simulink model "tg9"  (R2022a)
settings: Solver=ode15s  StartTime=0.0  StopTime=10  MaxStep=0.01  RelTol=1e-3
InitFcn:
  | mecha_param2
  | control_param0
values from neighbouring files (symbols this model uses):
  b0 = 0    [sim_IMMC.m]
  b1 = 1    [sim_IMMC.m]
  back0 = 0    [sim_IMMC.m]
  back1 = 0    [sim_IMMC.m]
  boff = 0    [sim_IMMC.m]
  bon = 0    [sim_IMMC.m]
  c = 0.05    [mecha_param2.m]
  c_jointstop = 0.3 / (pi/180)    (= 17.1887338539)    [mecha_param2.m]
  calctalus = sqrt((L_foot - (DJ1x_foot))^2 + (H_foot-r_cs)^2)    [mecha_param2.m]
  calctoes = sqrt((H_foot-r_cs)^2 + (DJ1x_foot)^2)    [mecha_param2.m]
  corrD = 0.001    [control_param0.m]
  DG_HAT = 0.35    [mecha_param2.m]
  DG_thigh = 0.28    [mecha_param2.m]
  DJ1x_foot = 0.16-r_cs    (= 0.135)    [mecha_param2.m]
  eref = 0.04    [mecha_param2.m]
  FmaxBFSH = 350    [mecha_param2.m]
  FmaxGAS = 1500    [mecha_param2.m]
  FmaxGLU = 1500    [mecha_param2.m]
  FmaxHAM = 3000    [mecha_param2.m]
  FmaxHFL = 2000    [mecha_param2.m]
  FmaxRF = 1200    [mecha_param2.m]
  FmaxSOL = 4000    [mecha_param2.m]
  FmaxTA = 800    [mecha_param2.m]
  FmaxVAS = 6000    [mecha_param2.m]
  g = 9.81    [mecha_param2.m]
  g0 = 0    [sim_IMMC.m]
  g1 = 0    [sim_IMMC.m]
  H_foot = 0.08    [mecha_param2.m]
  In_HAT = 3    [mecha_param2.m]
  In_shank = 0.05    [mecha_param2.m]
  In_thigh = 0.15    [mecha_param2.m]
  K = 5    [mecha_param2.m]
  knee_thigh = [0 0 -(L_thigh/2)]    [mecha_param2.m]
  Kpress = m_HAT * g / DeltaThRef    (= 104967)    [mecha_param2.m]
  L_foot = 0.2    [mecha_param2.m]
  L_HAT = 0.8    [mecha_param2.m]
  L_shank = 0.46    [mecha_param2.m]
  L_thigh = 0.46    [mecha_param2.m]
  LoHAM = table2array(mt('LoHAM', 1))    [control_param0.m]
  LoHFL = table2array(mt('LoHFL', 1))    [control_param0.m]
  longD = longD - corrD    (= 0.019)    [control_param0.m]
  loptBFSH = 0.12    [mecha_param2.m]
  loptGAS = 0.05    [mecha_param2.m]
  loptGLU = 0.11    [mecha_param2.m]
  loptHAM = 0.10    (= 0.1)    [mecha_param2.m]
  loptHFL = 0.11    [mecha_param2.m]
  loptRF = 0.08    [mecha_param2.m]
  loptSOL = 0.04    [mecha_param2.m]
  loptTA = 0.06    [mecha_param2.m]
  loptVAS = 0.08    [mecha_param2.m]
  LoTA = table2array(mt('LoTA', 1))    [control_param0.m]
  lslackBFSH = 0.10    (= 0.1)    [mecha_param2.m]
  lslackGAS = 0.40    (= 0.4)    [mecha_param2.m]
  lslackGLU = 0.13    [mecha_param2.m]
  lslackHAM = 0.31    [mecha_param2.m]
  lslackHFL = 0.10    (= 0.1)    [mecha_param2.m]
  lslackRF = 0.35    [mecha_param2.m]
  lslackSOL = 0.26    [mecha_param2.m]
  lslackTA = 0.24    [mecha_param2.m]
  lslackVAS = 0.23    [mecha_param2.m]
  m_HAT = 53.5    [mecha_param2.m]
  m_shank = 3.5    [mecha_param2.m]
  m_thigh = 8.5    [mecha_param2.m]
  midD = midD - corrD    (= 0.009)    [control_param0.m]
  N = 1.5    [mecha_param2.m]
  nonoff = 0    [control_param0.m]
  phi_a_low = (70) * (pi / 180)    (= 1.2217304764)    [mecha_param2.m]
  phi_a_up = (130) * (pi / 180)    (= 2.26892802759)    [mecha_param2.m]
  phi_dl = 180    [mecha_param2.m]
  phi_h = 230 * (pi / 180)    (= 4.01425727959)    [mecha_param2.m]
  phi_k = 175 * (pi / 180)    (= 3.05432619099)    [mecha_param2.m]
  phictoes = asind((DJ1y_foot-r_cs)/calctoes)    [mecha_param2.m]
  phimaxGASa = 100*pi/180    (= 1.74532925199)    [mecha_param2.m]
  phimaxGASk = 140*pi/180    (= 2.44346095279)    [mecha_param2.m]
  phimaxRFk = 165*pi/180    (= 2.87979326579)    [mecha_param2.m]
  phimaxSOL = 100*pi/180    (= 1.74532925199)    [mecha_param2.m]
  phimaxTA = 80*pi/180    (= 1.3962634016)    [mecha_param2.m]
  phimaxVAS = 165*pi/180    (= 2.87979326579)    [mecha_param2.m]
  phirefBFSH = 160*pi/180    (= 2.79252680319)    [mecha_param2.m]
  phirefGASa = 80*pi/180    (= 1.3962634016)    [mecha_param2.m]
  phirefGASk = 165*pi/180    (= 2.87979326579)    [mecha_param2.m]
  phirefGLU = 120*pi/180    (= 2.09439510239)    [mecha_param2.m]
  phirefHAMh = 150*pi/180    (= 2.61799387799)    [mecha_param2.m]
  phirefHAMk = 180*pi/180    (= 3.14159265359)    [mecha_param2.m]
  phirefHFL = 160*pi/180    (= 2.79252680319)    [mecha_param2.m]
  phirefRFh = 170*pi/180    (= 2.96705972839)    [mecha_param2.m]
  phirefRFk = 125*pi/180    (= 2.18166156499)    [mecha_param2.m]
  phirefSOL = 90*pi/180    (= 1.57079632679)    [mecha_param2.m]
  phirefTA = 110*pi/180    (= 1.91986217719)    [mecha_param2.m]
  phirefVAS = 120*pi/180    (= 2.09439510239)    [mecha_param2.m]
  phiScaleGASa = acos(rGASamin/rGASamax)/(phiminGASa-phimaxGASa)    [mecha_param2.m]
  phiScaleGASk = acos(rGASkmin/rGASkmax)/(phiminGASk-phimaxGASk)    [mecha_param2.m]
  phiScaleRFk = acos(rRFkmin/rRFkmax)/(phiminRFk-phimaxRFk)    [mecha_param2.m]
  phiScaleSOL = acos(rSOLmin/rSOLmax)/(phiminSOL-phimaxSOL)    [mecha_param2.m]
  phiScaleTA = acos(rTAmin/rTAmax)/(phiminTA-phimaxTA)    [mecha_param2.m]
  phiScaleVAS = acos(rVASmin/rVASmax)/(phiminVAS-phimaxVAS)    [mecha_param2.m]
  r1 = 0    [sim_IMMC.m]
  r_cs = 0.025    [mecha_param2.m]
  rBFSH = 0.04    [mecha_param2.m]
  rGASamax = 0.06    [mecha_param2.m]
  rGASkmax = 0.05    [mecha_param2.m]
  rGLU = 0.08    [mecha_param2.m]
  rHAMh = 0.08    [mecha_param2.m]
  rHAMk = 0.05    [mecha_param2.m]
  rHFL = 0.08    [mecha_param2.m]
  rhoBFSH = 0.7    [mecha_param2.m]
  rhoGASa = 0.7    [mecha_param2.m]
  rhoGASk = 0.7    [mecha_param2.m]
  rhoGLU = 0.5    [mecha_param2.m]
  rhoHAMh = 0.5    [mecha_param2.m]
  rhoHAMk = 0.5    [mecha_param2.m]
  rhoHFL = 0.5    [mecha_param2.m]
  rhoRFh = 0.3    [mecha_param2.m]
  rhoRFk = 0.5    [mecha_param2.m]
  rhoSOL = 0.5    [mecha_param2.m]
  rhoTA = 0.7    [mecha_param2.m]
  rhoVAS = 0.6    [mecha_param2.m]
  rRFh = 0.08    [mecha_param2.m]
  rRFkmax = 0.06    [mecha_param2.m]
  rSOLmax = 0.06    [mecha_param2.m]
  ... (+25 more)
undefined symbols (not defined in the file or in its folder): beta11, beta12, beta13, beta14, beta15, beta16, beta21, beta22, beta23, beta24, beta25, beta26, beta31, beta32, beta33, beta34, beta35, beta36, beta41, beta42, beta43, beta44, beta45, beta46, beta51, beta52, beta53, beta54, beta55, beta56, betab1, betab2, betab3, betab4, betab5, betab6, betap11, betap12, betap13, betap14, betap15, betap16, betap21, betap22, betap23, betap24, betap25, betap26, betap31, betap32, betap33, betap34, betap35, betap36, betap41, betap42, betap43, betap44, betap45, betap46 ... (+102)
libraries: sm_lib x89, simulink x72, nesl_utility x58, simulink_extras x18
(part 9 of 12)

== system tg9/Muscle Actuation Layer/L GLU/CE inverse force-velocity relation ==
  note: u(1) * (u(2)<=1)
  note: CE, inverse force-velocity relationship
  note: K*fv
  note: 1+K*fv
  note: fv-1
  Fv[Fmax] : Inport
  Constant{,1,3..4} (4 alike) : Constant
  Constant2 : Constant  Value=N
  Constant5 : Constant  Value=N
  Divide2 : Product  Inputs=/*
  Divide3 : Product  Inputs=*/
  Gain : Gain  Gain=K
  Gain2 : Gain  Gain=7.56*K
  Gain3 : Gain  Gain=1e-2
  Mux : Mux  Inputs=3
  Mux1 : Mux  Inputs=2
  Mux2 : Mux  Inputs=3
  Product : Product  Inputs=*/
  Sum : Sum  Inputs=|+-
  Sum1 : Sum  Inputs=++|
  Sum2 : Sum  Inputs=+|+
  Sum3 : Sum  Inputs=+|+
  Sum4 : Sum  Inputs=-+|
  Sum5 : Sum  Inputs=|-+
  Sum6 : Sum  Inputs=|++
  Sum7 : Sum  Inputs=+-|
  Sum8 : Sum  Inputs=|++
  excentric branch1 : Fcn  Expr=u(2) * (u(1)>1)*(u(1)<=u(3))
  excentric branch2 : Fcn  Expr=u(1) * (u(2)<=1)
  excentric branch3 : Fcn  Expr=u(3) * (u(2)>u(1))
  v[vmax] : Outport
  wires:
  Sum/1 -> Product/1
  Constant1/1 -> Sum/2, Sum1/1
  Gain/1 -> Sum1/2
  Sum1/1 -> Product/2
  Product/1 -> Mux1/1
  Mux1/1 -> excentric branch2/1
  excentric branch2/1 -> Sum3/1
  Sum3/1 -> v[vmax]/1
  Constant2/1 -> Sum5/2, Sum4/1
  Constant3/1 -> Sum5/1
  Sum5/1 -> Divide2/1
  Sum4/1 -> Gain3/1, Divide2/2
  Sum6/1 -> Divide3/1
  Constant/1 -> Sum7/1, Sum6/2
  Divide2/1 -> Gain2/1, Sum6/1
  Sum7/1 -> Divide3/2
  Gain2/1 -> Sum7/2
  Gain3/1 -> Sum8/1
  Constant4/1 -> Sum8/2
  Sum8/1 -> Mux/3
  Divide3/1 -> Mux2/2
  Constant5/1 -> Mux/1, Mux2/3
  Mux2/1 -> excentric branch1/1
  Mux/1 -> excentric branch3/1
  excentric branch1/1 -> Sum2/1
  excentric branch3/1 -> Sum2/2
  Sum2/1 -> Sum3/2
  Fv[Fmax]/1 -> Mux/2, Mux2/1, Mux1/2, Gain/1, Sum/1, Sum4/2

== system tg9/Muscle Actuation Layer/L GLU/PE force-length relation ==
  note: tendon reference strain, relative to lslack
  note: if lse > 1
  note: lce-1
  note: ((lce-1)/w)^2
  note: fpe, force-length relationship
  lce [lopt] : Inport
  Constant : Constant  Value=w
  Constant1 : Constant
  Math Function : Math  Operator=square
  Mux : Mux  Inputs=2
  Sum : Sum  Inputs=|+-
  excentric branch1 : Fcn  Expr=u(2) * (u(1)>1)
  relative strain : Product  Inputs=*/
  fpe [Fmax] : Outport
  wires:
  excentric branch1/1 -> fpe [Fmax]/1
  Mux/1 -> excentric branch1/1
  relative strain/1 -> Math Function/1
  Constant1/1 -> Sum/2
  Sum/1 -> relative strain/1
  lce [lopt]/1 -> Mux/1, Sum/1
  Constant/1 -> relative strain/2
  Math Function/1 -> Mux/2

== system tg9/Muscle Actuation Layer/L GLU/SE force-length relation ==
  note: fse, elastic force-length relationship
  note: tendon reference strain, relative to lslack
  note: e = (lse-lslack)/lslack;
      | e = lse[lslack]-1
  note: (e/eref)^2
  note: e>0 or lse>1
  lse [lslack] : Inport
  Constant : Constant  Value=eref
  Constant1 : Constant
  Math Function : Math  Operator=square
  Mux : Mux  Inputs=2
  Sum : Sum  Inputs=|+-
  excentric branch1 : Fcn  Expr=u(2)*(u(1)>1)
  relative strain : Product  Inputs=*/
  fse [Fmax] : Outport
  wires:
  lse [lslack]/1 -> Mux/1, Sum/1
  Sum/1 -> relative strain/1
  Constant1/1 -> Sum/2
  Constant/1 -> relative strain/2
  relative strain/1 -> Math Function/1
  Math Function/1 -> Mux/2
  Mux/1 -> excentric branch1/1
  excentric branch1/1 -> fse [Fmax]/1

== system tg9/Muscle Actuation Layer/L HAM/BE force-length relation ==
  note: reference compression
  note: if lce<1-w
  note: lce[lopt]-(1-w)
  note: ((lce+w-1)/(w/2))^2
  note: fbe, compression force-length relationship
  lce [lopt] : Inport
  Constant : Constant  Value=w/2
  Constant1 : Constant  Value=1-w
  Math Function : Math  Operator=square
  Mux : Mux  Inputs=2
  Sum : Sum  Inputs=|+-
  excentric branch1 : Fcn  Expr=u(2)*(u(1)<0)
  relative strain : Product  Inputs=*/
  fbe [Fmax] : Outport
  wires:
  excentric branch1/1 -> fbe [Fmax]/1
  Mux/1 -> excentric branch1/1
  relative strain/1 -> Math Function/1
  Constant1/1 -> Sum/2
  Sum/1 -> Mux/1, relative strain/1
  lce [lopt]/1 -> Sum/1
  Constant/1 -> relative strain/2
  Math Function/1 -> Mux/2

== system tg9/Muscle Actuation Layer/L HAM/CE force-length relation ==
  note: fce, force-length relationship
  note: lce-1
  note: |lce-1|
  note: |lce-1|/w
  note: (|lce-1|/w)^3
  lce [lopt] : Inport
  Abs : Abs  SaturateOnIntegerOverflow=off
  Constant : Constant
  Constant1 : Constant  Value=w
  Constant2 : Constant  Value=3
  Exp : Math
  Exp1 : Math  Operator=pow  SignedPower=on
  Gain : Gain  Gain=log(c)
  Sum : Sum  Inputs=|+-
  normalized position : Product  Inputs=*/
  fce [Fmax] : Outport
  wires:
  lce [lopt]/1 -> Sum/1
  Constant/1 -> Sum/2
  Constant1/1 -> normalized position/2
  Sum/1 -> Abs/1
  Abs/1 -> normalized position/1
  normalized position/1 -> Exp1/1
  Constant2/1 -> Exp1/2
  Exp1/1 -> Gain/1
  Gain/1 -> Exp/1
  Exp/1 -> fce [Fmax]/1

== system tg9/Muscle Actuation Layer/L HAM/CE inverse force-velocity relation ==
  note: u(1) * (u(2)<=1)
  note: CE, inverse force-velocity relationship
  note: K*fv
  note: 1+K*fv
  note: fv-1
  Fv[Fmax] : Inport
  Constant{,1,3..4} (4 alike) : Constant
  Constant2 : Constant  Value=N
  Constant5 : Constant  Value=N
  Divide2 : Product  Inputs=/*
  Divide3 : Product  Inputs=*/
  Gain : Gain  Gain=K
  Gain2 : Gain  Gain=7.56*K
  Gain3 : Gain  Gain=1e-2
  Mux : Mux  Inputs=3
  Mux1 : Mux  Inputs=2
  Mux2 : Mux  Inputs=3
  Product : Product  Inputs=*/
  Sum : Sum  Inputs=|+-
  Sum1 : Sum  Inputs=++|
  Sum2 : Sum  Inputs=+|+
  Sum3 : Sum  Inputs=+|+
  Sum4 : Sum  Inputs=-+|
  Sum5 : Sum  Inputs=|-+
  Sum6 : Sum  Inputs=|++
  Sum7 : Sum  Inputs=+-|
  Sum8 : Sum  Inputs=|++
  excentric branch1 : Fcn  Expr=u(2) * (u(1)>1)*(u(1)<=u(3))
  excentric branch2 : Fcn  Expr=u(1) * (u(2)<=1)
  excentric branch3 : Fcn  Expr=u(3) * (u(2)>u(1))
  v[vmax] : Outport
  wires:
  Sum/1 -> Product/1
  Constant1/1 -> Sum/2, Sum1/1
  Gain/1 -> Sum1/2
  Sum1/1 -> Product/2
  Product/1 -> Mux1/1
  Mux1/1 -> excentric branch2/1
  excentric branch2/1 -> Sum3/1
  Sum3/1 -> v[vmax]/1
  Constant2/1 -> Sum5/2, Sum4/1
  Constant3/1 -> Sum5/1
  Sum5/1 -> Divide2/1
  Sum4/1 -> Gain3/1, Divide2/2
  Sum6/1 -> Divide3/1
  Constant/1 -> Sum7/1, Sum6/2
  Divide2/1 -> Gain2/1, Sum6/1
  Sum7/1 -> Divide3/2
  Gain2/1 -> Sum7/2
  Gain3/1 -> Sum8/1
  Constant4/1 -> Sum8/2
  Sum8/1 -> Mux/3
  Divide3/1 -> Mux2/2
  Constant5/1 -> Mux/1, Mux2/3
  Mux2/1 -> excentric branch1/1
  Mux/1 -> excentric branch3/1
  excentric branch1/1 -> Sum2/1
  excentric branch3/1 -> Sum2/2
  Sum2/1 -> Sum3/2
  Fv[Fmax]/1 -> Mux/2, Mux2/1, Mux1/2, Gain/1, Sum/1, Sum4/2

== system tg9/Muscle Actuation Layer/L HAM/PE force-length relation ==
  note: tendon reference strain, relative to lslack
  note: if lse > 1
  note: lce-1
  note: ((lce-1)/w)^2
  note: fpe, force-length relationship
  lce [lopt] : Inport
  Constant : Constant  Value=w
  Constant1 : Constant
  Math Function : Math  Operator=square
  Mux : Mux  Inputs=2
  Sum : Sum  Inputs=|+-
  excentric branch1 : Fcn  Expr=u(2) * (u(1)>1)
  relative strain : Product  Inputs=*/
  fpe [Fmax] : Outport
  wires:
  excentric branch1/1 -> fpe [Fmax]/1
  Mux/1 -> excentric branch1/1
  relative strain/1 -> Math Function/1
  Constant1/1 -> Sum/2
  Sum/1 -> relative strain/1
  lce [lopt]/1 -> Mux/1, Sum/1
  Constant/1 -> relative strain/2
  Math Function/1 -> Mux/2

== system tg9/Muscle Actuation Layer/L HAM/SE force-length relation ==
  note: fse, elastic force-length relationship
  note: tendon reference strain, relative to lslack
  note: e = (lse-lslack)/lslack;
      | e = lse[lslack]-1
  note: (e/eref)^2
  note: e>0 or lse>1
  lse [lslack] : Inport
  Constant : Constant  Value=eref
  Constant1 : Constant
  Math Function : Math  Operator=square
  Mux : Mux  Inputs=2
  Sum : Sum  Inputs=|+-
  excentric branch1 : Fcn  Expr=u(2)*(u(1)>1)
  relative strain : Product  Inputs=*/
  fse [Fmax] : Outport
  wires:
  lse [lslack]/1 -> Mux/1, Sum/1
  Sum/1 -> relative strain/1
  Constant1/1 -> Sum/2
  Constant/1 -> relative strain/2
  relative strain/1 -> Math Function/1
  Math Function/1 -> Mux/2
  Mux/1 -> excentric branch1/1
  excentric branch1/1 -> fse [Fmax]/1

== system tg9/Muscle Actuation Layer/L HFL/BE force-length relation ==
  note: reference compression
  note: if lce<1-w
  note: lce[lopt]-(1-w)
  note: ((lce+w-1)/(w/2))^2
  note: fbe, compression force-length relationship
  lce [lopt] : Inport
  Constant : Constant  Value=w/2
  Constant1 : Constant  Value=1-w
  Math Function : Math  Operator=square
  Mux : Mux  Inputs=2
  Sum : Sum  Inputs=|+-
  excentric branch1 : Fcn  Expr=u(2)*(u(1)<0)
  relative strain : Product  Inputs=*/
  fbe [Fmax] : Outport
  wires:
  excentric branch1/1 -> fbe [Fmax]/1
  Mux/1 -> excentric branch1/1
  relative strain/1 -> Math Function/1
  Constant1/1 -> Sum/2
  Sum/1 -> Mux/1, relative strain/1
  lce [lopt]/1 -> Sum/1
  Constant/1 -> relative strain/2
  Math Function/1 -> Mux/2

== system tg9/Muscle Actuation Layer/L HFL/CE force-length relation ==
  note: fce, force-length relationship
  note: lce-1
  note: |lce-1|
  note: |lce-1|/w
  note: (|lce-1|/w)^3
  lce [lopt] : Inport
  Abs : Abs  SaturateOnIntegerOverflow=off
  Constant : Constant
  Constant1 : Constant  Value=w
  Constant2 : Constant  Value=3
  Exp : Math
  Exp1 : Math  Operator=pow  SignedPower=on
  Gain : Gain  Gain=log(c)
  Sum : Sum  Inputs=|+-
  normalized position : Product  Inputs=*/
  fce [Fmax] : Outport
  wires:
  lce [lopt]/1 -> Sum/1
  Constant/1 -> Sum/2
  Constant1/1 -> normalized position/2
  Sum/1 -> Abs/1
  Abs/1 -> normalized position/1
  normalized position/1 -> Exp1/1
  Constant2/1 -> Exp1/2
  Exp1/1 -> Gain/1
  Gain/1 -> Exp/1
  Exp/1 -> fce [Fmax]/1

== system tg9/Muscle Actuation Layer/L HFL/CE inverse force-velocity relation ==
  note: u(1) * (u(2)<=1)
  note: CE, inverse force-velocity relationship
  note: K*fv
  note: 1+K*fv
  note: fv-1
  Fv[Fmax] : Inport
  Constant{,1,3..4} (4 alike) : Constant
  Constant2 : Constant  Value=N
  Constant5 : Constant  Value=N
  Divide2 : Product  Inputs=/*
  Divide3 : Product  Inputs=*/
  Gain : Gain  Gain=K
  Gain2 : Gain  Gain=7.56*K
  Gain3 : Gain  Gain=1e-2
  Mux : Mux  Inputs=3
  Mux1 : Mux  Inputs=2
  Mux2 : Mux  Inputs=3
  Product : Product  Inputs=*/
  Sum : Sum  Inputs=|+-
  Sum1 : Sum  Inputs=++|
  Sum2 : Sum  Inputs=+|+
  Sum3 : Sum  Inputs=+|+
  Sum4 : Sum  Inputs=-+|
  Sum5 : Sum  Inputs=|-+
  Sum6 : Sum  Inputs=|++
  Sum7 : Sum  Inputs=+-|
  Sum8 : Sum  Inputs=|++
  excentric branch1 : Fcn  Expr=u(2) * (u(1)>1)*(u(1)<=u(3))
  excentric branch2 : Fcn  Expr=u(1) * (u(2)<=1)
  excentric branch3 : Fcn  Expr=u(3) * (u(2)>u(1))
  v[vmax] : Outport
  wires:
  Sum/1 -> Product/1
  Constant1/1 -> Sum/2, Sum1/1
  Gain/1 -> Sum1/2
  Sum1/1 -> Product/2
  Product/1 -> Mux1/1
  Mux1/1 -> excentric branch2/1
  excentric branch2/1 -> Sum3/1
  Sum3/1 -> v[vmax]/1
  Constant2/1 -> Sum5/2, Sum4/1
  Constant3/1 -> Sum5/1
  Sum5/1 -> Divide2/1
  Sum4/1 -> Gain3/1, Divide2/2
  Sum6/1 -> Divide3/1
  Constant/1 -> Sum7/1, Sum6/2
  Divide2/1 -> Gain2/1, Sum6/1
  Sum7/1 -> Divide3/2
  Gain2/1 -> Sum7/2
  Gain3/1 -> Sum8/1
  Constant4/1 -> Sum8/2
  Sum8/1 -> Mux/3
  Divide3/1 -> Mux2/2
  Constant5/1 -> Mux/1, Mux2/3
  Mux2/1 -> excentric branch1/1
  Mux/1 -> excentric branch3/1
  excentric branch1/1 -> Sum2/1
  excentric branch3/1 -> Sum2/2
  Sum2/1 -> Sum3/2
  Fv[Fmax]/1 -> Mux/2, Mux2/1, Mux1/2, Gain/1, Sum/1, Sum4/2

== system tg9/Muscle Actuation Layer/L HFL/PE force-length relation ==
  note: tendon reference strain, relative to lslack
  note: if lse > 1
  note: lce-1
  note: ((lce-1)/w)^2
  note: fpe, force-length relationship
  lce [lopt] : Inport
  Constant : Constant  Value=w
  Constant1 : Constant
  Math Function : Math  Operator=square
  Mux : Mux  Inputs=2
  Sum : Sum  Inputs=|+-
  excentric branch1 : Fcn  Expr=u(2) * (u(1)>1)
  relative strain : Product  Inputs=*/
  fpe [Fmax] : Outport
  wires:
  excentric branch1/1 -> fpe [Fmax]/1
  Mux/1 -> excentric branch1/1
  relative strain/1 -> Math Function/1
  Constant1/1 -> Sum/2
  Sum/1 -> relative strain/1
  lce [lopt]/1 -> Mux/1, Sum/1
  Constant/1 -> relative strain/2
  Math Function/1 -> Mux/2

== system tg9/Muscle Actuation Layer/L HFL/SE force-length relation ==
  note: fse, elastic force-length relationship
  note: tendon reference strain, relative to lslack
  note: e = (lse-lslack)/lslack;
      | e = lse[lslack]-1
  note: (e/eref)^2
  note: e>0 or lse>1
  lse [lslack] : Inport
  Constant : Constant  Value=eref
  Constant1 : Constant
  Math Function : Math  Operator=square
  Mux : Mux  Inputs=2
  Sum : Sum  Inputs=|+-
  excentric branch1 : Fcn  Expr=u(2)*(u(1)>1)
  relative strain : Product  Inputs=*/
  fse [Fmax] : Outport
  wires:
  lse [lslack]/1 -> Mux/1, Sum/1
  Sum/1 -> relative strain/1
  Constant1/1 -> Sum/2
  Constant/1 -> relative strain/2
  relative strain/1 -> Math Function/1
  Math Function/1 -> Mux/2
  Mux/1 -> excentric branch1/1
  excentric branch1/1 -> fse [Fmax]/1

== system tg9/Muscle Actuation Layer/L RF/BE force-length relation ==
  note: fbe, compression force-length relationship
  note: ((lce+w-1)/(w/2))^2
  note: lce[lopt]-(1-w)
  note: if lce<1-w
  note: reference compression
  lce [lopt] : Inport
  Constant : Constant  Value=w/2
  Constant1 : Constant  Value=1-w
  Math Function : Math  Operator=square
  Mux : Mux  Inputs=2
  Sum : Sum  Inputs=|+-
  excentric branch1 : Fcn  Expr=u(2)*(u(1)<0)
  relative strain : Product  Inputs=*/
  fbe [Fmax] : Outport
  wires:
  Math Function/1 -> Mux/2
  Constant/1 -> relative strain/2
  lce [lopt]/1 -> Sum/1
  Sum/1 -> relative strain/1, Mux/1
  Constant1/1 -> Sum/2
  relative strain/1 -> Math Function/1
  Mux/1 -> excentric branch1/1
  excentric branch1/1 -> fbe [Fmax]/1

== system tg9/Muscle Actuation Layer/L RF/CE force-length relation ==
  note: (|lce-1|/w)^3
  note: |lce-1|/w
  note: |lce-1|
  note: lce-1
  note: fce, force-length relationship
  lce [lopt] : Inport
  Abs : Abs  SaturateOnIntegerOverflow=off
  Constant : Constant
  Constant1 : Constant  Value=w
  Constant2 : Constant  Value=3
  Exp : Math
  Exp1 : Math  Operator=pow  SignedPower=on
  Gain : Gain  Gain=log(c)
  Sum : Sum  Inputs=|+-
  normalized position : Product  Inputs=*/
  fce [Fmax] : Outport
  wires:
  Exp/1 -> fce [Fmax]/1
  Gain/1 -> Exp/1
  Exp1/1 -> Gain/1
  Constant2/1 -> Exp1/2
  normalized position/1 -> Exp1/1
  Abs/1 -> normalized position/1
  Sum/1 -> Abs/1
  Constant1/1 -> normalized position/2
  Constant/1 -> Sum/2
  lce [lopt]/1 -> Sum/1

== system tg9/Muscle Actuation Layer/L RF/CE inverse force-velocity relation ==
  note: fv-1
  note: 1+K*fv
  note: K*fv
  note: CE, inverse force-velocity relationship
  note: u(1) * (u(2)<=1)
  Fv[Fmax] : Inport
  Constant{,1,3..4} (4 alike) : Constant
  Constant2 : Constant  Value=N
  Constant5 : Constant  Value=N
  Divide2 : Product  Inputs=/*
  Divide3 : Product  Inputs=*/
  Gain : Gain  Gain=K
  Gain2 : Gain  Gain=7.56*K
  Gain3 : Gain  Gain=1e-2
  Mux : Mux  Inputs=3
  Mux1 : Mux  Inputs=2
  Mux2 : Mux  Inputs=3
  Product : Product  Inputs=*/
  Sum : Sum  Inputs=|+-
  Sum1 : Sum  Inputs=++|
  Sum2 : Sum  Inputs=+|+
  Sum3 : Sum  Inputs=+|+
  Sum4 : Sum  Inputs=-+|
  Sum5 : Sum  Inputs=|-+
  Sum6 : Sum  Inputs=|++
  Sum7 : Sum  Inputs=+-|
  Sum8 : Sum  Inputs=|++
  excentric branch1 : Fcn  Expr=u(2) * (u(1)>1)*(u(1)<=u(3))
  excentric branch2 : Fcn  Expr=u(1) * (u(2)<=1)
  excentric branch3 : Fcn  Expr=u(3) * (u(2)>u(1))
  v[vmax] : Outport
  wires:
  Fv[Fmax]/1 -> Sum4/2, Sum/1, Gain/1, Mux1/2, Mux2/1, Mux/2
  Sum2/1 -> Sum3/2
  excentric branch3/1 -> Sum2/2
  excentric branch1/1 -> Sum2/1
  Mux/1 -> excentric branch3/1
  Mux2/1 -> excentric branch1/1
  Constant5/1 -> Mux2/3, Mux/1
  Divide3/1 -> Mux2/2
  Sum8/1 -> Mux/3
  Constant4/1 -> Sum8/2
  Gain3/1 -> Sum8/1
  Gain2/1 -> Sum7/2
  Sum7/1 -> Divide3/2
  Divide2/1 -> Sum6/1, Gain2/1
  Constant/1 -> Sum6/2, Sum7/1
  Sum6/1 -> Divide3/1
  Sum4/1 -> Divide2/2, Gain3/1
  Sum5/1 -> Divide2/1
  Constant3/1 -> Sum5/1
  Constant2/1 -> Sum4/1, Sum5/2
  Sum3/1 -> v[vmax]/1
  excentric branch2/1 -> Sum3/1
  Mux1/1 -> excentric branch2/1
  Product/1 -> Mux1/1
  Sum1/1 -> Product/2
  Gain/1 -> Sum1/2
  Constant1/1 -> Sum1/1, Sum/2
  Sum/1 -> Product/1

== system tg9/Muscle Actuation Layer/L RF/PE force-length relation ==
  note: fpe, force-length relationship
  note: ((lce-1)/w)^2
  note: lce-1
  note: if lse > 1
  note: tendon reference strain, relative to lslack
  lce [lopt] : Inport
  Constant : Constant  Value=w
  Constant1 : Constant
  Math Function : Math  Operator=square
  Mux : Mux  Inputs=2
  Sum : Sum  Inputs=|+-
  excentric branch1 : Fcn  Expr=u(2) * (u(1)>1)
  relative strain : Product  Inputs=*/
  fpe [Fmax] : Outport
  wires:
  Math Function/1 -> Mux/2
  Constant/1 -> relative strain/2
  lce [lopt]/1 -> Sum/1, Mux/1
  Sum/1 -> relative strain/1
  Constant1/1 -> Sum/2
  relative strain/1 -> Math Function/1
  Mux/1 -> excentric branch1/1
  excentric branch1/1 -> fpe [Fmax]/1

== system tg9/Muscle Actuation Layer/L RF/SE force-length relation ==
  note: e>0 or lse>1
  note: (e/eref)^2
  note: e = (lse-lslack)/lslack;
      | e = lse[lslack]-1
  note: tendon reference strain, relative to lslack
  note: fse, elastic force-length relationship
  lse [lslack] : Inport
  Constant : Constant  Value=eref
  Constant1 : Constant
  Math Function : Math  Operator=square
  Mux : Mux  Inputs=2
  Sum : Sum  Inputs=|+-
  excentric branch1 : Fcn  Expr=u(2)*(u(1)>1)
  relative strain : Product  Inputs=*/
  fse [Fmax] : Outport
  wires:
  excentric branch1/1 -> fse [Fmax]/1
  Mux/1 -> excentric branch1/1
  Math Function/1 -> Mux/2
  relative strain/1 -> Math Function/1
  Constant/1 -> relative strain/2
  Constant1/1 -> Sum/2
  Sum/1 -> relative strain/1
  lse [lslack]/1 -> Sum/1, Mux/1

== system tg9/Muscle Actuation Layer/L SOL/BE force-length relation ==
  note: reference compression
  note: if lce<1-w
  note: lce[lopt]-(1-w)
  note: ((lce+w-1)/(w/2))^2
  note: fbe, compression force-length relationship
  lce [lopt] : Inport
  Constant : Constant  Value=w/2
  Constant1 : Constant  Value=1-w
  Math Function : Math  Operator=square
  Mux : Mux  Inputs=2
  Sum : Sum  Inputs=|+-
  excentric branch1 : Fcn  Expr=u(2)*(u(1)<0)
  relative strain : Product  Inputs=*/
  fbe [Fmax] : Outport
  wires:
  excentric branch1/1 -> fbe [Fmax]/1
  Mux/1 -> excentric branch1/1
  relative strain/1 -> Math Function/1
  Constant1/1 -> Sum/2
  Sum/1 -> Mux/1, relative strain/1
  lce [lopt]/1 -> Sum/1
  Constant/1 -> relative strain/2
  Math Function/1 -> Mux/2

== system tg9/Muscle Actuation Layer/L SOL/CE force-length relation ==
  note: fce, force-length relationship
  note: lce-1
  note: |lce-1|
  note: |lce-1|/w
  note: (|lce-1|/w)^3
  lce [lopt] : Inport
  Abs : Abs  SaturateOnIntegerOverflow=off
  Constant : Constant
  Constant1 : Constant  Value=w
  Constant2 : Constant  Value=3
  Exp : Math
  Exp1 : Math  Operator=pow  SignedPower=on
  Gain : Gain  Gain=log(c)
  Sum : Sum  Inputs=|+-
  normalized position : Product  Inputs=*/
  fce [Fmax] : Outport
  wires:
  lce [lopt]/1 -> Sum/1
  Constant/1 -> Sum/2
  Constant1/1 -> normalized position/2
  Sum/1 -> Abs/1
  Abs/1 -> normalized position/1
  normalized position/1 -> Exp1/1
  Constant2/1 -> Exp1/2
  Exp1/1 -> Gain/1
  Gain/1 -> Exp/1
  Exp/1 -> fce [Fmax]/1

== system tg9/Muscle Actuation Layer/L SOL/CE inverse force-velocity relation ==
  note: u(1) * (u(2)<=1)
  note: CE, inverse force-velocity relationship
  note: K*fv
  note: 1+K*fv
  note: fv-1
  Fv[Fmax] : Inport
  Constant{,1,3..4} (4 alike) : Constant
  Constant2 : Constant  Value=N
  Constant5 : Constant  Value=N
  Divide2 : Product  Inputs=/*
  Divide3 : Product  Inputs=*/
  Gain : Gain  Gain=K
  Gain2 : Gain  Gain=7.56*K
  Gain3 : Gain  Gain=1e-2
  Mux : Mux  Inputs=3
  Mux1 : Mux  Inputs=2
  Mux2 : Mux  Inputs=3
  Product : Product  Inputs=*/
  Sum : Sum  Inputs=|+-
  Sum1 : Sum  Inputs=++|
  Sum2 : Sum  Inputs=+|+
  Sum3 : Sum  Inputs=+|+
  Sum4 : Sum  Inputs=-+|
  Sum5 : Sum  Inputs=|-+
  Sum6 : Sum  Inputs=|++
  Sum7 : Sum  Inputs=+-|
  Sum8 : Sum  Inputs=|++
  excentric branch1 : Fcn  Expr=u(2) * (u(1)>1)*(u(1)<=u(3))
  excentric branch2 : Fcn  Expr=u(1) * (u(2)<=1)
  excentric branch3 : Fcn  Expr=u(3) * (u(2)>u(1))
  v[vmax] : Outport
  wires:
  Sum/1 -> Product/1
  Constant1/1 -> Sum/2, Sum1/1
  Gain/1 -> Sum1/2
  Sum1/1 -> Product/2
  Product/1 -> Mux1/1
  Mux1/1 -> excentric branch2/1
  excentric branch2/1 -> Sum3/1
  Sum3/1 -> v[vmax]/1
  Constant2/1 -> Sum5/2, Sum4/1
  Constant3/1 -> Sum5/1
  Sum5/1 -> Divide2/1
  Sum4/1 -> Gain3/1, Divide2/2
  Sum6/1 -> Divide3/1
  Constant/1 -> Sum7/1, Sum6/2
  Divide2/1 -> Gain2/1, Sum6/1
  Sum7/1 -> Divide3/2
  Gain2/1 -> Sum7/2
  Gain3/1 -> Sum8/1
  Constant4/1 -> Sum8/2
  Sum8/1 -> Mux/3
  Divide3/1 -> Mux2/2
  Constant5/1 -> Mux/1, Mux2/3
  Mux2/1 -> excentric branch1/1
  Mux/1 -> excentric branch3/1
  excentric branch1/1 -> Sum2/1
  excentric branch3/1 -> Sum2/2
  Sum2/1 -> Sum3/2
  Fv[Fmax]/1 -> Mux/2, Mux2/1, Mux1/2, Gain/1, Sum/1, Sum4/2

== system tg9/Muscle Actuation Layer/L SOL/PE force-length relation ==
  note: tendon reference strain, relative to lslack
  note: if lse > 1
  note: lce-1
  note: ((lce-1)/w)^2
  note: fpe, force-length relationship
  lce [lopt] : Inport
  Constant : Constant  Value=w
  Constant1 : Constant
  Math Function : Math  Operator=square
  Mux : Mux  Inputs=2
  Sum : Sum  Inputs=|+-
  excentric branch1 : Fcn  Expr=u(2) * (u(1)>1)
  relative strain : Product  Inputs=*/
  fpe [Fmax] : Outport
  wires:
  excentric branch1/1 -> fpe [Fmax]/1
  Mux/1 -> excentric branch1/1
  relative strain/1 -> Math Function/1
  Constant1/1 -> Sum/2
  Sum/1 -> relative strain/1
  lce [lopt]/1 -> Mux/1, Sum/1
  Constant/1 -> relative strain/2
  Math Function/1 -> Mux/2

== system tg9/Muscle Actuation Layer/L SOL/SE force-length relation ==
  note: fse, elastic force-length relationship
  note: tendon reference strain, relative to lslack
  note: e = (lse-lslack)/lslack;
      | e = lse[lslack]-1
  note: (e/eref)^2
  note: e>0 or lse>1
  lse [lslack] : Inport
  Constant : Constant  Value=eref
  Constant1 : Constant
  Math Function : Math  Operator=square
  Mux : Mux  Inputs=2
  Sum : Sum  Inputs=|+-
  excentric branch1 : Fcn  Expr=u(2)*(u(1)>1)
  relative strain : Product  Inputs=*/
  fse [Fmax] : Outport
  wires:
  lse [lslack]/1 -> Mux/1, Sum/1
  Sum/1 -> relative strain/1
  Constant1/1 -> Sum/2
  Constant/1 -> relative strain/2
  relative strain/1 -> Math Function/1
  Math Function/1 -> Mux/2
  Mux/1 -> excentric branch1/1
  excentric branch1/1 -> fse [Fmax]/1

== system tg9/Muscle Actuation Layer/L TA/BE force-length relation ==
  note: reference compression
  note: if lce<1-w
  note: lce[lopt]-(1-w)
  note: ((lce+w-1)/(w/2))^2
  note: fbe, compression force-length relationship
  lce [lopt] : Inport
  Constant : Constant  Value=w/2
  Constant1 : Constant  Value=1-w
  Math Function : Math  Operator=square
  Mux : Mux  Inputs=2
  Sum : Sum  Inputs=|+-
  excentric branch1 : Fcn  Expr=u(2)*(u(1)<0)
  relative strain : Product  Inputs=*/
  fbe [Fmax] : Outport
  wires:
  excentric branch1/1 -> fbe [Fmax]/1
  Mux/1 -> excentric branch1/1
  relative strain/1 -> Math Function/1
  Constant1/1 -> Sum/2
  Sum/1 -> Mux/1, relative strain/1
  lce [lopt]/1 -> Sum/1
  Constant/1 -> relative strain/2
  Math Function/1 -> Mux/2

== system tg9/Muscle Actuation Layer/L TA/CE force-length relation ==
  note: fce, force-length relationship
  note: lce-1
  note: |lce-1|
  note: |lce-1|/w
  note: (|lce-1|/w)^3
  lce [lopt] : Inport
  Abs : Abs  SaturateOnIntegerOverflow=off
  Constant : Constant
  Constant1 : Constant  Value=w
  Constant2 : Constant  Value=3
  Exp : Math
  Exp1 : Math  Operator=pow  SignedPower=on
  Gain : Gain  Gain=log(c)
  Sum : Sum  Inputs=|+-
  normalized position : Product  Inputs=*/
  fce [Fmax] : Outport
  wires:
  lce [lopt]/1 -> Sum/1
  Constant/1 -> Sum/2
  Constant1/1 -> normalized position/2
  Sum/1 -> Abs/1
  Abs/1 -> normalized position/1
  normalized position/1 -> Exp1/1
  Constant2/1 -> Exp1/2
  Exp1/1 -> Gain/1
  Gain/1 -> Exp/1
  Exp/1 -> fce [Fmax]/1

== system tg9/Muscle Actuation Layer/L TA/CE inverse force-velocity relation ==
  note: u(1) * (u(2)<=1)
  note: CE, inverse force-velocity relationship
  note: K*fv
  note: 1+K*fv
  note: fv-1
  Fv[Fmax] : Inport
  Constant{,1,3..4} (4 alike) : Constant
  Constant2 : Constant  Value=N
  Constant5 : Constant  Value=N
  Divide2 : Product  Inputs=/*
  Divide3 : Product  Inputs=*/
  Gain : Gain  Gain=K
  Gain2 : Gain  Gain=7.56*K
  Gain3 : Gain  Gain=1e-2
  Mux : Mux  Inputs=3
  Mux1 : Mux  Inputs=2
  Mux2 : Mux  Inputs=3
  Product : Product  Inputs=*/
  Sum : Sum  Inputs=|+-
  Sum1 : Sum  Inputs=++|
  Sum2 : Sum  Inputs=+|+
  Sum3 : Sum  Inputs=+|+
  Sum4 : Sum  Inputs=-+|
  Sum5 : Sum  Inputs=|-+
  Sum6 : Sum  Inputs=|++
  Sum7 : Sum  Inputs=+-|
  Sum8 : Sum  Inputs=|++
  excentric branch1 : Fcn  Expr=u(2) * (u(1)>1)*(u(1)<=u(3))
  excentric branch2 : Fcn  Expr=u(1) * (u(2)<=1)
  excentric branch3 : Fcn  Expr=u(3) * (u(2)>u(1))
  v[vmax] : Outport
  wires:
  Sum/1 -> Product/1
  Constant1/1 -> Sum/2, Sum1/1
  Gain/1 -> Sum1/2
  Sum1/1 -> Product/2
  Product/1 -> Mux1/1
  Mux1/1 -> excentric branch2/1
  excentric branch2/1 -> Sum3/1
  Sum3/1 -> v[vmax]/1
  Constant2/1 -> Sum5/2, Sum4/1
  Constant3/1 -> Sum5/1
  Sum5/1 -> Divide2/1
  Sum4/1 -> Gain3/1, Divide2/2
  Sum6/1 -> Divide3/1
  Constant/1 -> Sum7/1, Sum6/2
  Divide2/1 -> Gain2/1, Sum6/1
  Sum7/1 -> Divide3/2
  Gain2/1 -> Sum7/2
  Gain3/1 -> Sum8/1
  Constant4/1 -> Sum8/2
  Sum8/1 -> Mux/3
  Divide3/1 -> Mux2/2
  Constant5/1 -> Mux/1, Mux2/3
  Mux2/1 -> excentric branch1/1
  Mux/1 -> excentric branch3/1
  excentric branch1/1 -> Sum2/1
  excentric branch3/1 -> Sum2/2
  Sum2/1 -> Sum3/2
  Fv[Fmax]/1 -> Mux/2, Mux2/1, Mux1/2, Gain/1, Sum/1, Sum4/2

== system tg9/Muscle Actuation Layer/L TA/PE force-length relation ==
  note: tendon reference strain, relative to lslack
  note: if lse > 1
  note: lce-1
  note: ((lce-1)/w)^2
  note: fpe, force-length relationship
  lce [lopt] : Inport
  Constant : Constant  Value=w
  Constant1 : Constant
  Math Function : Math  Operator=square
  Mux : Mux  Inputs=2
  Sum : Sum  Inputs=|+-
  excentric branch1 : Fcn  Expr=u(2) * (u(1)>1)
  relative strain : Product  Inputs=*/
  fpe [Fmax] : Outport
  wires:
  excentric branch1/1 -> fpe [Fmax]/1
  Mux/1 -> excentric branch1/1
  relative strain/1 -> Math Function/1
  Constant1/1 -> Sum/2
  Sum/1 -> relative strain/1
  lce [lopt]/1 -> Mux/1, Sum/1
  Constant/1 -> relative strain/2
  Math Function/1 -> Mux/2

== system tg9/Muscle Actuation Layer/L TA/SE force-length relation ==
  note: fse, elastic force-length relationship
  note: tendon reference strain, relative to lslack
  note: e = (lse-lslack)/lslack;
      | e = lse[lslack]-1
  note: (e/eref)^2
  note: e>0 or lse>1
  lse [lslack] : Inport
  Constant : Constant  Value=eref
  Constant1 : Constant
  Math Function : Math  Operator=square
  Mux : Mux  Inputs=2
  Sum : Sum  Inputs=|+-
  excentric branch1 : Fcn  Expr=u(2)*(u(1)>1)
  relative strain : Product  Inputs=*/
  fse [Fmax] : Outport
  wires:
  lse [lslack]/1 -> Mux/1, Sum/1
  Sum/1 -> relative strain/1
  Constant1/1 -> Sum/2
  Constant/1 -> relative strain/2
  relative strain/1 -> Math Function/1
  Math Function/1 -> Mux/2
  Mux/1 -> excentric branch1/1
  excentric branch1/1 -> fse [Fmax]/1

== system tg9/Muscle Actuation Layer/L VAS/BE force-length relation ==
  note: reference compression
  note: if lce<1-w
  note: lce[lopt]-(1-w)
  note: ((lce+w-1)/(w/2))^2
  note: fbe, compression force-length relationship
  lce [lopt] : Inport
  Constant : Constant  Value=w/2
  Constant1 : Constant  Value=1-w
  Math Function : Math  Operator=square
  Mux : Mux  Inputs=2
  Sum : Sum  Inputs=|+-
  excentric branch1 : Fcn  Expr=u(2)*(u(1)<0)
  relative strain : Product  Inputs=*/
  fbe [Fmax] : Outport
  wires:
  excentric branch1/1 -> fbe [Fmax]/1
  Mux/1 -> excentric branch1/1
  relative strain/1 -> Math Function/1
  Constant1/1 -> Sum/2
  Sum/1 -> Mux/1, relative strain/1
  lce [lopt]/1 -> Sum/1
  Constant/1 -> relative strain/2
  Math Function/1 -> Mux/2

== system tg9/Muscle Actuation Layer/L VAS/CE force-length relation ==
  note: fce, force-length relationship
  note: lce-1
  note: |lce-1|
  note: |lce-1|/w
  note: (|lce-1|/w)^3
  lce [lopt] : Inport
  Abs : Abs  SaturateOnIntegerOverflow=off
  Constant : Constant
  Constant1 : Constant  Value=w
  Constant2 : Constant  Value=3
  Exp : Math
  Exp1 : Math  Operator=pow  SignedPower=on
  Gain : Gain  Gain=log(c)
  Sum : Sum  Inputs=|+-
  normalized position : Product  Inputs=*/
  fce [Fmax] : Outport
  wires:
  lce [lopt]/1 -> Sum/1
  Constant/1 -> Sum/2
  Constant1/1 -> normalized position/2
  Sum/1 -> Abs/1
  Abs/1 -> normalized position/1
  normalized position/1 -> Exp1/1
  Constant2/1 -> Exp1/2
  Exp1/1 -> Gain/1
  Gain/1 -> Exp/1
  Exp/1 -> fce [Fmax]/1

== system tg9/Muscle Actuation Layer/L VAS/CE inverse force-velocity relation ==
  note: u(1) * (u(2)<=1)
  note: CE, inverse force-velocity relationship
  note: K*fv
  note: 1+K*fv
  note: fv-1
  Fv[Fmax] : Inport
  Constant{,1,3..4} (4 alike) : Constant
  Constant2 : Constant  Value=N
  Constant5 : Constant  Value=N
  Divide2 : Product  Inputs=/*
  Divide3 : Product  Inputs=*/
  Gain : Gain  Gain=K
  Gain2 : Gain  Gain=7.56*K
  Gain3 : Gain  Gain=1e-2
  Mux : Mux  Inputs=3
  Mux1 : Mux  Inputs=2
  Mux2 : Mux  Inputs=3
  Product : Product  Inputs=*/
  Sum : Sum  Inputs=|+-
  Sum1 : Sum  Inputs=++|
  Sum2 : Sum  Inputs=+|+
  Sum3 : Sum  Inputs=+|+
  Sum4 : Sum  Inputs=-+|
  Sum5 : Sum  Inputs=|-+
  Sum6 : Sum  Inputs=|++
  Sum7 : Sum  Inputs=+-|
  Sum8 : Sum  Inputs=|++
  excentric branch1 : Fcn  Expr=u(2) * (u(1)>1)*(u(1)<=u(3))
  excentric branch2 : Fcn  Expr=u(1) * (u(2)<=1)
  excentric branch3 : Fcn  Expr=u(3) * (u(2)>u(1))
  v[vmax] : Outport
  wires:
  Sum/1 -> Product/1
  Constant1/1 -> Sum/2, Sum1/1
  Gain/1 -> Sum1/2
  Sum1/1 -> Product/2
  Product/1 -> Mux1/1
  Mux1/1 -> excentric branch2/1
  excentric branch2/1 -> Sum3/1
  Sum3/1 -> v[vmax]/1
  Constant2/1 -> Sum5/2, Sum4/1
  Constant3/1 -> Sum5/1
  Sum5/1 -> Divide2/1
  Sum4/1 -> Gain3/1, Divide2/2
  Sum6/1 -> Divide3/1
  Constant/1 -> Sum7/1, Sum6/2
  Divide2/1 -> Gain2/1, Sum6/1
  Sum7/1 -> Divide3/2
  Gain2/1 -> Sum7/2
  Gain3/1 -> Sum8/1
  Constant4/1 -> Sum8/2
  Sum8/1 -> Mux/3
  Divide3/1 -> Mux2/2
  Constant5/1 -> Mux/1, Mux2/3
  Mux2/1 -> excentric branch1/1
  Mux/1 -> excentric branch3/1
  excentric branch1/1 -> Sum2/1
  excentric branch3/1 -> Sum2/2
  Sum2/1 -> Sum3/2
  Fv[Fmax]/1 -> Mux/2, Mux2/1, Mux1/2, Gain/1, Sum/1, Sum4/2

== system tg9/Muscle Actuation Layer/L VAS/PE force-length relation ==
  note: tendon reference strain, relative to lslack
  note: if lse > 1
  note: lce-1
  note: ((lce-1)/w)^2
  note: fpe, force-length relationship
  lce [lopt] : Inport
  Constant : Constant  Value=w
  Constant1 : Constant
  Math Function : Math  Operator=square
  Mux : Mux  Inputs=2
  Sum : Sum  Inputs=|+-
  excentric branch1 : Fcn  Expr=u(2) * (u(1)>1)
  relative strain : Product  Inputs=*/
  fpe [Fmax] : Outport
  wires:
  excentric branch1/1 -> fpe [Fmax]/1
  Mux/1 -> excentric branch1/1
  relative strain/1 -> Math Function/1
  Constant1/1 -> Sum/2
  Sum/1 -> relative strain/1
  lce [lopt]/1 -> Mux/1, Sum/1
  Constant/1 -> relative strain/2
  Math Function/1 -> Mux/2

== system tg9/Muscle Actuation Layer/L VAS/SE force-length relation ==
  note: fse, elastic force-length relationship
  note: tendon reference strain, relative to lslack
  note: e = (lse-lslack)/lslack;
      | e = lse[lslack]-1
  note: (e/eref)^2
  note: e>0 or lse>1
  lse [lslack] : Inport
  Constant : Constant  Value=eref
  Constant1 : Constant
  Math Function : Math  Operator=square
  Mux : Mux  Inputs=2
  Sum : Sum  Inputs=|+-
  excentric branch1 : Fcn  Expr=u(2)*(u(1)>1)
  relative strain : Product  Inputs=*/
  fse [Fmax] : Outport
  wires:
  lse [lslack]/1 -> Mux/1, Sum/1
  Sum/1 -> relative strain/1
  Constant1/1 -> Sum/2
  Constant/1 -> relative strain/2
  relative strain/1 -> Math Function/1
  Math Function/1 -> Mux/2
  Mux/1 -> excentric branch1/1
  excentric branch1/1 -> fse [Fmax]/1

== system tg9/Muscle Actuation Layer/R BFSH/BE force-length relation ==
  note: fbe, compression force-length relationship
  note: ((lce+w-1)/(w/2))^2
  note: lce[lopt]-(1-w)
  note: if lce<1-w
  note: reference compression
  lce [lopt] : Inport
  Constant : Constant  Value=w/2
  Constant1 : Constant  Value=1-w
  Math Function : Math  Operator=square
  Mux : Mux  Inputs=2
  Sum : Sum  Inputs=|+-
  excentric branch1 : Fcn  Expr=u(2)*(u(1)<0)
  relative strain : Product  Inputs=*/
  fbe [Fmax] : Outport
  wires:
  Math Function/1 -> Mux/2
  Constant/1 -> relative strain/2
  lce [lopt]/1 -> Sum/1
  Sum/1 -> relative strain/1, Mux/1
  Constant1/1 -> Sum/2
  relative strain/1 -> Math Function/1
  Mux/1 -> excentric branch1/1
  excentric branch1/1 -> fbe [Fmax]/1

== system tg9/Muscle Actuation Layer/R BFSH/CE force-length relation ==
  note: (|lce-1|/w)^3
  note: |lce-1|/w
  note: |lce-1|
  note: lce-1
  note: fce, force-length relationship
  lce [lopt] : Inport
  Abs : Abs  SaturateOnIntegerOverflow=off
  Constant : Constant
  Constant1 : Constant  Value=w
  Constant2 : Constant  Value=3
  Exp : Math
  Exp1 : Math  Operator=pow  SignedPower=on
  Gain : Gain  Gain=log(c)
  Sum : Sum  Inputs=|+-
  normalized position : Product  Inputs=*/
  fce [Fmax] : Outport
  wires:
  Exp/1 -> fce [Fmax]/1
  Gain/1 -> Exp/1
  Exp1/1 -> Gain/1
  Constant2/1 -> Exp1/2
  normalized position/1 -> Exp1/1
  Abs/1 -> normalized position/1
  Sum/1 -> Abs/1
  Constant1/1 -> normalized position/2
  Constant/1 -> Sum/2
  lce [lopt]/1 -> Sum/1

== system tg9/Muscle Actuation Layer/R BFSH/CE inverse force-velocity relation ==
  note: fv-1
  note: 1+K*fv
  note: K*fv
  note: CE, inverse force-velocity relationship
  note: u(1) * (u(2)<=1)
  Fv[Fmax] : Inport
  Constant{,1,3..4} (4 alike) : Constant
  Constant2 : Constant  Value=N
  Constant5 : Constant  Value=N
  Divide2 : Product  Inputs=/*
  Divide3 : Product  Inputs=*/
  Gain : Gain  Gain=K
  Gain2 : Gain  Gain=7.56*K
  Gain3 : Gain  Gain=1e-2
  Mux : Mux  Inputs=3
  Mux1 : Mux  Inputs=2
  Mux2 : Mux  Inputs=3
  Product : Product  Inputs=*/
  Sum : Sum  Inputs=|+-
  Sum1 : Sum  Inputs=++|
  Sum2 : Sum  Inputs=+|+
  Sum3 : Sum  Inputs=+|+
  Sum4 : Sum  Inputs=-+|
  Sum5 : Sum  Inputs=|-+
  Sum6 : Sum  Inputs=|++
  Sum7 : Sum  Inputs=+-|
  Sum8 : Sum  Inputs=|++
  excentric branch1 : Fcn  Expr=u(2) * (u(1)>1)*(u(1)<=u(3))
  excentric branch2 : Fcn  Expr=u(1) * (u(2)<=1)
  excentric branch3 : Fcn  Expr=u(3) * (u(2)>u(1))
  v[vmax] : Outport
  wires:
  Fv[Fmax]/1 -> Sum4/2, Sum/1, Gain/1, Mux1/2, Mux2/1, Mux/2
  Sum2/1 -> Sum3/2
  excentric branch3/1 -> Sum2/2
  excentric branch1/1 -> Sum2/1
  Mux/1 -> excentric branch3/1
  Mux2/1 -> excentric branch1/1
  Constant5/1 -> Mux2/3, Mux/1
  Divide3/1 -> Mux2/2
  Sum8/1 -> Mux/3
  Constant4/1 -> Sum8/2
  Gain3/1 -> Sum8/1
  Gain2/1 -> Sum7/2
  Sum7/1 -> Divide3/2
  Divide2/1 -> Sum6/1, Gain2/1
  Constant/1 -> Sum6/2, Sum7/1
  Sum6/1 -> Divide3/1
  Sum4/1 -> Divide2/2, Gain3/1
  Sum5/1 -> Divide2/1
  Constant3/1 -> Sum5/1
  Constant2/1 -> Sum4/1, Sum5/2
  Sum3/1 -> v[vmax]/1
  excentric branch2/1 -> Sum3/1
  Mux1/1 -> excentric branch2/1
  Product/1 -> Mux1/1
  Sum1/1 -> Product/2
  Gain/1 -> Sum1/2
  Constant1/1 -> Sum1/1, Sum/2
  Sum/1 -> Product/1

== system tg9/Muscle Actuation Layer/R BFSH/PE force-length relation ==
  note: fpe, force-length relationship
  note: ((lce-1)/w)^2
  note: lce-1
  note: if lse > 1
  note: tendon reference strain, relative to lslack
  lce [lopt] : Inport
  Constant : Constant  Value=w
  Constant1 : Constant
  Math Function : Math  Operator=square
  Mux : Mux  Inputs=2
  Sum : Sum  Inputs=|+-
  excentric branch1 : Fcn  Expr=u(2) * (u(1)>1)
  relative strain : Product  Inputs=*/
  fpe [Fmax] : Outport
  wires:
  Math Function/1 -> Mux/2
  Constant/1 -> relative strain/2
  lce [lopt]/1 -> Sum/1, Mux/1
  Sum/1 -> relative strain/1
  Constant1/1 -> Sum/2
  relative strain/1 -> Math Function/1
  Mux/1 -> excentric branch1/1
  excentric branch1/1 -> fpe [Fmax]/1

== system tg9/Muscle Actuation Layer/R BFSH/SE force-length relation ==
  note: e>0 or lse>1
  note: (e/eref)^2
  note: e = (lse-lslack)/lslack;
      | e = lse[lslack]-1
  note: tendon reference strain, relative to lslack
  note: fse, elastic force-length relationship
  lse [lslack] : Inport
  Constant : Constant  Value=eref
  Constant1 : Constant
  Math Function : Math  Operator=square
  Mux : Mux  Inputs=2
  Sum : Sum  Inputs=|+-
  excentric branch1 : Fcn  Expr=u(2)*(u(1)>1)
  relative strain : Product  Inputs=*/
  fse [Fmax] : Outport
  wires:
  excentric branch1/1 -> fse [Fmax]/1
  Mux/1 -> excentric branch1/1
  Math Function/1 -> Mux/2
  relative strain/1 -> Math Function/1
  Constant/1 -> relative strain/2
  Constant1/1 -> Sum/2
  Sum/1 -> relative strain/1
  lse [lslack]/1 -> Sum/1, Mux/1

== system tg9/Muscle Actuation Layer/R GAS/BE force-length relation ==
  note: reference compression
  note: if lce<1-w
  note: lce[lopt]-(1-w)
  note: ((lce+w-1)/(w/2))^2
  note: fbe, compression force-length relationship
  lce [lopt] : Inport
  Constant : Constant  Value=w/2
  Constant1 : Constant  Value=1-w
  Math Function : Math  Operator=square
  Mux : Mux  Inputs=2
  Sum : Sum  Inputs=|+-
  excentric branch1 : Fcn  Expr=u(2)*(u(1)<0)
  relative strain : Product  Inputs=*/
  fbe [Fmax] : Outport
  wires:
  excentric branch1/1 -> fbe [Fmax]/1
  Mux/1 -> excentric branch1/1
  relative strain/1 -> Math Function/1
  Constant1/1 -> Sum/2
  Sum/1 -> Mux/1, relative strain/1
  lce [lopt]/1 -> Sum/1
  Constant/1 -> relative strain/2
  Math Function/1 -> Mux/2

== system tg9/Muscle Actuation Layer/R GAS/CE force-length relation ==
  note: fce, force-length relationship
  note: lce-1
  note: |lce-1|
  note: |lce-1|/w
  note: (|lce-1|/w)^3
  lce [lopt] : Inport
  Abs : Abs  SaturateOnIntegerOverflow=off
  Constant : Constant
  Constant1 : Constant  Value=w
  Constant2 : Constant  Value=3
  Exp : Math
  Exp1 : Math  Operator=pow  SignedPower=on
  Gain : Gain  Gain=log(c)
  Sum : Sum  Inputs=|+-
  normalized position : Product  Inputs=*/
  fce [Fmax] : Outport
  wires:
  lce [lopt]/1 -> Sum/1
  Constant/1 -> Sum/2
  Constant1/1 -> normalized position/2
  Sum/1 -> Abs/1
  Abs/1 -> normalized position/1
  normalized position/1 -> Exp1/1
  Constant2/1 -> Exp1/2
  Exp1/1 -> Gain/1
  Gain/1 -> Exp/1
  Exp/1 -> fce [Fmax]/1

== system tg9/Muscle Actuation Layer/R GAS/CE inverse force-velocity relation ==
  note: u(1) * (u(2)<=1)
  note: CE, inverse force-velocity relationship
  note: K*fv
  note: 1+K*fv
  note: fv-1
  Fv[Fmax] : Inport
  Constant{,1,3..4} (4 alike) : Constant
  Constant2 : Constant  Value=N
  Constant5 : Constant  Value=N
  Divide2 : Product  Inputs=/*
  Divide3 : Product  Inputs=*/
  Gain : Gain  Gain=K
  Gain2 : Gain  Gain=7.56*K
  Gain3 : Gain  Gain=1e-2
  Mux : Mux  Inputs=3
  Mux1 : Mux  Inputs=2
  Mux2 : Mux  Inputs=3
  Product : Product  Inputs=*/
  Sum : Sum  Inputs=|+-
  Sum1 : Sum  Inputs=++|
  Sum2 : Sum  Inputs=+|+
  Sum3 : Sum  Inputs=+|+
  Sum4 : Sum  Inputs=-+|
  Sum5 : Sum  Inputs=|-+
  Sum6 : Sum  Inputs=|++
  Sum7 : Sum  Inputs=+-|
  Sum8 : Sum  Inputs=|++
  excentric branch1 : Fcn  Expr=u(2) * (u(1)>1)*(u(1)<=u(3))
  excentric branch2 : Fcn  Expr=u(1) * (u(2)<=1)
  excentric branch3 : Fcn  Expr=u(3) * (u(2)>u(1))
  v[vmax] : Outport
  wires:
  Sum/1 -> Product/1
  Constant1/1 -> Sum/2, Sum1/1
  Gain/1 -> Sum1/2
  Sum1/1 -> Product/2
  Product/1 -> Mux1/1
  Mux1/1 -> excentric branch2/1
  excentric branch2/1 -> Sum3/1
  Sum3/1 -> v[vmax]/1
  Constant2/1 -> Sum5/2, Sum4/1
  Constant3/1 -> Sum5/1
  Sum5/1 -> Divide2/1
  Sum4/1 -> Gain3/1, Divide2/2
  Sum6/1 -> Divide3/1
  Constant/1 -> Sum7/1, Sum6/2
  Divide2/1 -> Gain2/1, Sum6/1
  Sum7/1 -> Divide3/2
  Gain2/1 -> Sum7/2
  Gain3/1 -> Sum8/1
  Constant4/1 -> Sum8/2
  Sum8/1 -> Mux/3
  Divide3/1 -> Mux2/2
  Constant5/1 -> Mux/1, Mux2/3
  Mux2/1 -> excentric branch1/1
  Mux/1 -> excentric branch3/1
  excentric branch1/1 -> Sum2/1
  excentric branch3/1 -> Sum2/2
  Sum2/1 -> Sum3/2
  Fv[Fmax]/1 -> Mux/2, Mux2/1, Mux1/2, Gain/1, Sum/1, Sum4/2

== system tg9/Muscle Actuation Layer/R GAS/PE force-length relation ==
  note: tendon reference strain, relative to lslack
  note: if lse > 1
  note: lce-1
  note: ((lce-1)/w)^2
  note: fpe, force-length relationship
  lce [lopt] : Inport
  Constant : Constant  Value=w
  Constant1 : Constant
  Math Function : Math  Operator=square
  Mux : Mux  Inputs=2
  Sum : Sum  Inputs=|+-
  excentric branch1 : Fcn  Expr=u(2) * (u(1)>1)
  relative strain : Product  Inputs=*/
  fpe [Fmax] : Outport
  wires:
  excentric branch1/1 -> fpe [Fmax]/1
  Mux/1 -> excentric branch1/1
  relative strain/1 -> Math Function/1
  Constant1/1 -> Sum/2
  Sum/1 -> relative strain/1
  lce [lopt]/1 -> Mux/1, Sum/1
  Constant/1 -> relative strain/2
  Math Function/1 -> Mux/2

== system tg9/Muscle Actuation Layer/R GAS/SE force-length relation ==
  note: fse, elastic force-length relationship
  note: tendon reference strain, relative to lslack
  note: e = (lse-lslack)/lslack;
      | e = lse[lslack]-1
  note: (e/eref)^2
  note: e>0 or lse>1
  lse [lslack] : Inport
  Constant : Constant  Value=eref
  Constant1 : Constant
  Math Function : Math  Operator=square
  Mux : Mux  Inputs=2
  Sum : Sum  Inputs=|+-
  excentric branch1 : Fcn  Expr=u(2)*(u(1)>1)
  relative strain : Product  Inputs=*/
  fse [Fmax] : Outport
  wires:
  lse [lslack]/1 -> Mux/1, Sum/1
  Sum/1 -> relative strain/1
  Constant1/1 -> Sum/2
  Constant/1 -> relative strain/2
  relative strain/1 -> Math Function/1
  Math Function/1 -> Mux/2
  Mux/1 -> excentric branch1/1
  excentric branch1/1 -> fse [Fmax]/1

== system tg9/Muscle Actuation Layer/R GLU/BE force-length relation ==
  note: reference compression
  note: if lce<1-w
  note: lce[lopt]-(1-w)
  note: ((lce+w-1)/(w/2))^2
  note: fbe, compression force-length relationship
  lce [lopt] : Inport
  Constant : Constant  Value=w/2
  Constant1 : Constant  Value=1-w
  Math Function : Math  Operator=square
  Mux : Mux  Inputs=2
  Sum : Sum  Inputs=|+-
  excentric branch1 : Fcn  Expr=u(2)*(u(1)<0)
  relative strain : Product  Inputs=*/
  fbe [Fmax] : Outport
  wires:
  excentric branch1/1 -> fbe [Fmax]/1
  Mux/1 -> excentric branch1/1
  relative strain/1 -> Math Function/1
  Constant1/1 -> Sum/2
  Sum/1 -> Mux/1, relative strain/1
  lce [lopt]/1 -> Sum/1
  Constant/1 -> relative strain/2
  Math Function/1 -> Mux/2

== system tg9/Muscle Actuation Layer/R GLU/CE force-length relation ==
  note: fce, force-length relationship
  note: lce-1
  note: |lce-1|
  note: |lce-1|/w
  note: (|lce-1|/w)^3
  lce [lopt] : Inport
  Abs : Abs  SaturateOnIntegerOverflow=off
  Constant : Constant
  Constant1 : Constant  Value=w
  Constant2 : Constant  Value=3
  Exp : Math
  Exp1 : Math  Operator=pow  SignedPower=on
  Gain : Gain  Gain=log(c)
  Sum : Sum  Inputs=|+-
  normalized position : Product  Inputs=*/
  fce [Fmax] : Outport
  wires:
  lce [lopt]/1 -> Sum/1
  Constant/1 -> Sum/2
  Constant1/1 -> normalized position/2
  Sum/1 -> Abs/1
  Abs/1 -> normalized position/1
  normalized position/1 -> Exp1/1
  Constant2/1 -> Exp1/2
  Exp1/1 -> Gain/1
  Gain/1 -> Exp/1
  Exp/1 -> fce [Fmax]/1
